simulink model "mas508_cw34_example1"  (R2021b)
settings: Solver=FixedStepAuto  StartTime=0.0  StopTime=2  FixedStep=1e-3  RelTol=1e-3
settings Model: Creator=rtavares  LastModifiedBy=faisala
settings SolverCC: AlgebraicLoopSolver=TrustRegion
settings DataIOCC: ReturnWorkspaceOutputs=off
settings DebuggingCC: SFMachineParentedDataDiag=warning

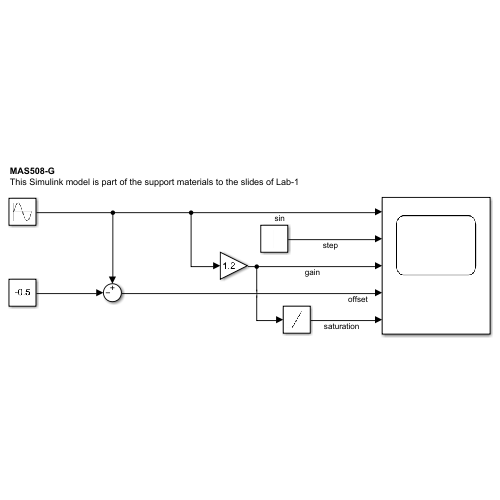
[thumbnail: Simulink's stored preview of the top-level diagram]
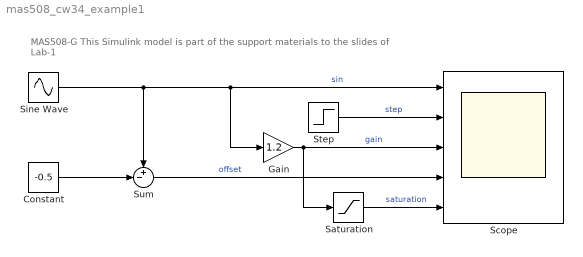
== system mas508_cw34_example1 ==
  note: MAS508-G
      | This Simulink model is part of the support materials to the slides of Lab-1
  Constant : Constant  Value=-0.5
  Gain : Gain  Gain=1.2
  Saturation : Saturate  UpperLimit=1  LowerLimit=-1
  Scope : Scope  NumInputPorts=5
  Sine Wave : Sin  Frequency=2*pi*3  SampleTime=0
  Step : Step  Time=0.5  SampleTime=0
  Sum : Sum  Inputs=+-|
  wires:
  Sine Wave/1 -> Scope/1, Gain/1, Sum/1  "sin"
  Step/1 -> Scope/2  "step"
  Gain/1 -> Saturation/1, Scope/3  "gain"
  Constant/1 -> Sum/2
  Sum/1 -> Scope/4  "offset"
  Saturation/1 -> Scope/5  "saturation"
